simulink model "fft_inputs_equal_size_test"  (Simulink 7.2)
settings: Solver=VariableStepDiscrete  StartTime=0.0  StopTime=64  RelTol=1e-3
libraries: xbsIndex_r4 x249, casper_library_misc x24
(part 1 of 3)
settings Model: Creator=User  LastModifiedBy=root
settings OptimizationCC: InitFltsAndDblsToZero=on
settings DebuggingCC: SaveWithDisabledLinksMsg=none  SaveWithParameterizedLinksMsg=none

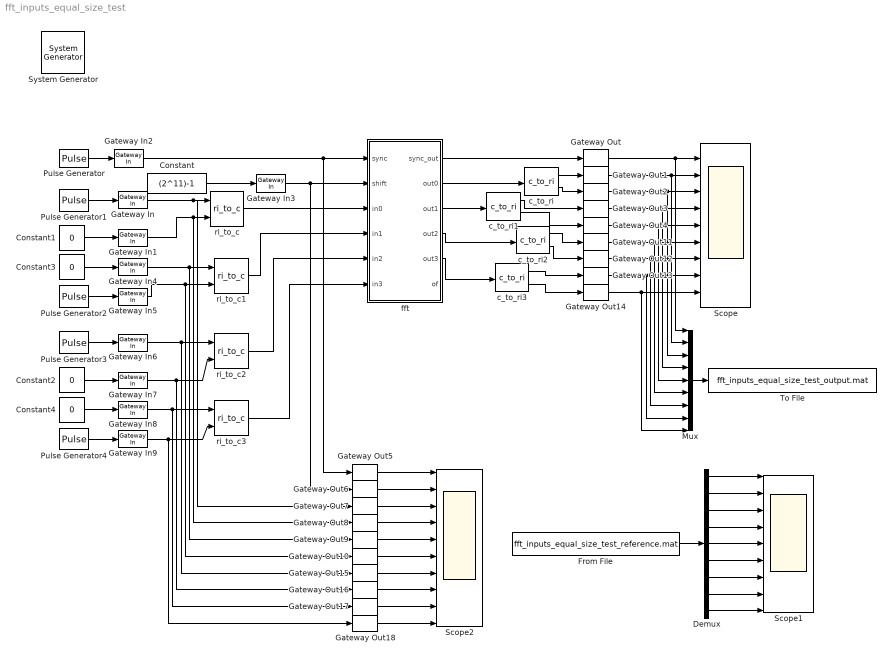
== system fft_inputs_equal_size_test ==
  " System Generator" : xbsIndex_r4/ System Generator  Tag=genX  SystemSampleTime=-1  xilinxfamily=Virtex4  part=xc4vsx35  speed=-10  package=ff668  synthesis_tool=XST  clock_wrapper=Clock Enables  directory=./netlist  testbench=off  simulink_period=1  sysclk_period=100  dcm_input_clock_period=100  incr_netlist=off  trim_vbits=Everywhere in SubSystem  dbl_ovrd=According to Block Masks  core_generation=According to Block Masks  run_coregen=off  deprecated_control=off  eval_field=0  block_type=sysgen
      settings: block_version=10.1.1
  Constant : Constant  Value=(2^11)-1  OutDataType=sfix(16)  OutScaling=2^0
  Constant{1..4} (4 alike) : Constant  Value=0  OutDataType=sfix(16)  OutScaling=2^0
  Demux : Demux  Outputs=9
  From File : FromFile  FileName=fft_inputs_equal_size_test_reference.mat  SampleTime=1
  Gateway In{,1,4..9} (8 alike) : xbsIndex_r4/Gateway In  arith_type="Signed  (2's comp)"  n_bits=8  bin_pt=7  quantization=Truncate  overflow=Wrap  period=1  dbl_ovrd=off  timing_constraint=None  locs_specified=off  LOCs={}  hdl_port=on  block_type=gatewayin
      settings: infoedit="Gateway in block.  Converts inputs of type Simulink integer, double and fixed point to  Xilinx fixed point type.<P><P>Hardware notes:  In hardware these blocks become top level input ports."  block_version=10.1.1
  Gateway In2 : xbsIndex_r4/Gateway In  arith_type=Boolean  n_bits=18  bin_pt=17  quantization=Truncate  overflow=Wrap  period=1  dbl_ovrd=off  timing_constraint=None  locs_specified=off  LOCs={}  hdl_port=on  block_type=gatewayin
      settings: infoedit="Gateway in block.  Converts inputs of type Simulink integer, double and fixed point to  Xilinx fixed point type.<P><P>Hardware notes:  In hardware these blocks become top level input ports."  block_version=10.1.1
  Gateway In3 : xbsIndex_r4/Gateway In  arith_type=Unsigned  n_bits=11  bin_pt=0  quantization=Truncate  overflow=Wrap  period=1  dbl_ovrd=off  timing_constraint=None  locs_specified=off  LOCs={}  hdl_port=on  block_type=gatewayin
      settings: infoedit="Gateway in block.  Converts inputs of type Simulink integer, double and fixed point to  Xilinx fixed point type.<P><P>Hardware notes:  In hardware these blocks become top level input ports."  block_version=10.1.1
  Gateway Out{,1..18} (19 alike) : xbsIndex_r4/Gateway Out  hdl_port=on  timing_constraint=None  locs_specified=off  LOCs={}  block_type=gatewayout
      settings: infoedit="Gateway out block.  Converts Xilinx fixed point inputs into ouputs of type Simulink integer, double, or fixed point.<P><P>Hardware notes:  In hardware these blocks become top level output ports or are discarded, depending on how they are configured."  block_version=10.1.1
  Mux : Mux  Inputs=9
  Pulse Generator : DiscretePulseGenerator  Period=2^4  PhaseDelay=11
  Pulse Generator1 : DiscretePulseGenerator  Period=2^2  PhaseDelay=13
  Pulse Generator2 : DiscretePulseGenerator  Period=2^3  PhaseDelay=13
  Pulse Generator3 : DiscretePulseGenerator  Period=2^2  PhaseDelay=13
  Pulse Generator4 : DiscretePulseGenerator  Period=2^3  PhaseDelay=13
  Scope : Scope  NumInputPorts=9
      settings: YMin=-1~0~0~-5~-5~-5~-5~-5~-5  YMax=2~1~1~5~5~5~5~5~5
  Scope1 : Scope  NumInputPorts=9
      settings: YMin=-1~0~0~-5~-5~-5~-5~-5~-5  YMax=2~1~1~5~5~5~5~5~5
  Scope2 : Scope  NumInputPorts=10
      settings: YMin=-1~0~0~-5~-5~-5~-5~-5~-5~-5  YMax=2~1~1~5~5~5~5~5~5~5  SaveName=ScopeData2
  To File : ToFile  Filename=fft_inputs_equal_size_test_output.mat  MatrixName=output
  c_to_ri{,1..3} (4 alike) : casper_library_misc/c_to_ri  SystemSampleTime=-1  n_bits=8  bin_pt=7
      settings: AttributesFormatString=8_7 r/i
  fft : Subsystem  AncestorBlock=casper_library_ffts/fft  mask(fft){FFTSize=2, input_bit_width=8, coeff_bit_width=8, n_inputs=2, quantization=Truncate, overflow=Wrap, add_latency=2, mult_latency=3, bram_latency=1, conv_latency=2, arch=Virtex2Pro, opt_target=multipliers, coeffs_bit_limit=8, delays_bit_limit=8, specify_mult=on, mult_spec=[1                                      2], dsp48_adders=off}
      mask prompts: FFTSize "Size of FFT: (2^?)"; input_bit_width "Input/Output Bit Width"; coeff_bit_width "Coefficient Bit Width"; n_inputs "Number of Simultaneous Inputs: (2^?)"; quantization "Quantization Behavior"; overflow "Overflow Behavior"; add_latency "Add Latency"; mult_latency "Mult Latency"; bram_latency "BRAM Latency"; conv_latency "Convert latency"; arch "Architecture"; opt_target "Use less"; coeffs_bit_limit "Number bits above which to store stage's coefficients in BRAM (2^? bits)"; delays_bit_limit "Number bits above which to store stage's delays in BRAM (2^? bits)"; specify_mult "Specify multiplier use (behavioral HDL if not specified)"; mult_spec "Multiplier specification (0=core, 1=embedded, 2=behavioural) (left=1st stage)"; dsp48_adders "DSP48 adders in butterfly"
      mask init:
      | fft_init(gcb,...
      |     'FFTSize', FFTSize, ...
      |     'input_bit_width', input_bit_width, ...
      |     'coeff_bit_width', coeff_bit_width, ...
      |     'n_inputs', n_inputs, ...
      |     'quantization', quantization, ...
      |     'overflow', overflow, ...
      |     'add_latency', add_latency, ...
      |     'mult_latency', mult_latency, ...
      |     'bram_latency', bram_latency, ...
      |     'conv_latency', conv_latency, ...
      |     'arch', arch, ...
      |     'opt_target', opt_target, ...
      |     'coeffs_bit_limit', coeffs_bit_limit, ...
      |     'delays_bit_limit', delays_bit_limit, ...
      |     'specify_mult', specify_mult, ...
      |     'mult_spec', mult_spec, ...
      |     'dsp48_adders', dsp48_adders);
      settings: AttributesFormatString=|
      | 2 stages
      | (8,8)
      | Truncate
      | Wrap
      mask Help: eval('xlWeb(''http://casper.berkeley.edu/wiki/Fft'')')
      mask StyleString: edit,edit,edit,edit,popup(Truncate|Round  (unbiased: +/- Inf)|Round  (unbiased: Even Values)),popup(Wrap|Saturate|Error),edit,edit,edit,edit,popup(Virtex2Pro|Virtex5),popup(logic|multipliers),edit,edit,checkbox,edit,checkbox
      mask CallbackString:
      | % fft_size = eval(get_param(gcb, 'FFTSize'));
      | % old_vec = eval(get_param(gcb, 'mult_spec'));
      | 
      | % vec = 2.*ones(1,fft_size);
      | % old_size = length(old_vec);
      | 
      | % if(old_size <= fft_size), size = old_size;
      | % else, size = fft_size;
      | % end
      | 
      | % for n = 1:size, vec(n) = old_vec(n); end
      | % set_param(gcb, 'mult_spec', mat2str(vec));||||||||||fft_callback_arch(gcb);||||specify_mult = get_param(gcb,'specify_mult');
      | visibs = get_param(gcb, 'MaskVisibilities');
      | if( strcmp(specify_mult,'off')), visibs{16} = 'off';
      | else visibs{16} = 'on';
      | end
      | set_param(gcb, 'MaskVisibilities', visibs);
      | 
      | |% vec = eval( get_param(gcb, 'mult_spec'));
      | % vec_size = length(vec);
      | % fft_size = eval( get_param(gcb, 'FFTSize'));
      | % new_vec = 2.*ones(1, fft_size);
      | 
      | % if(vec_size <= fft_size), size = vec_size;
      | % else size = fft_size;
      | % end
      | 
      | % for n=1:size,
      | %    new_vec(n) = vec(n);
      | % end
      | % set_param(gcb, 'mult_spec', mat2str(new_vec));|fft_callback_dsp48_adders(gcb);
  ri_to_c{,1..3} (4 alike) : casper_library_misc/ri_to_c  SystemSampleTime=-1
  wires:
  Pulse Generator/1 -> Gateway In2/1
  Gateway In2/1 -> Gateway Out5/1, fft/1(sync)
  Constant/1 -> Gateway In3/1
  Gateway In3/1 -> Gateway Out6/1, fft/2(shift)
  fft/1(sync_out) -> Gateway Out/1
  fft/2(out0) -> c_to_ri/1
  c_to_ri/1 -> Gateway Out1/1
  c_to_ri/2 -> Gateway Out2/1
  c_to_ri1/2 -> Gateway Out4/1
  fft/3(out1) -> c_to_ri1/1
  c_to_ri1/1 -> Gateway Out3/1
  Gateway Out/1 -> Scope/1, Mux/1
  Pulse Generator1/1 -> Gateway In/1
  Gateway In/1 -> ri_to_c/1, Gateway Out7/1
  Constant1/1 -> Gateway In1/1
  Gateway In1/1 -> ri_to_c/2, Gateway Out8/1
  Gateway In4/1 -> ri_to_c1/1, Gateway Out9/1
  Gateway In5/1 -> ri_to_c1/2, Gateway Out10/1
  Gateway Out1/1 -> Scope/2, Mux/2
  Gateway Out2/1 -> Scope/3, Mux/3
  Mux/1 -> To File/1
  Demux/1 -> Scope1/1
  Demux/2 -> Scope1/2
  Demux/3 -> Scope1/3
  Demux/4 -> Scope1/4
  Demux/5 -> Scope1/5
  Gateway Out5/1 -> Scope2/1
  Gateway Out6/1 -> Scope2/2
  Gateway Out7/1 -> Scope2/3
  Gateway Out8/1 -> Scope2/4
  Gateway Out9/1 -> Scope2/5
  Gateway Out10/1 -> Scope2/6
  Constant3/1 -> Gateway In4/1
  Pulse Generator2/1 -> Gateway In5/1
  Pulse Generator3/1 -> Gateway In6/1
  Constant2/1 -> Gateway In7/1
  Constant4/1 -> Gateway In8/1
  Pulse Generator4/1 -> Gateway In9/1
  Gateway In6/1 -> ri_to_c2/1, Gateway Out15/1
  Gateway In7/1 -> ri_to_c2/2, Gateway Out16/1
  Gateway In8/1 -> ri_to_c3/1, Gateway Out17/1
  Gateway In9/1 -> ri_to_c3/2, Gateway Out18/1
  ri_to_c/1 -> fft/3(in0)
  ri_to_c1/1 -> fft/4(in1)
  ri_to_c2/1 -> fft/5(in2)
  ri_to_c3/1 -> fft/6(in3)
  fft/4(out2) -> c_to_ri2/1
  fft/5(out3) -> c_to_ri3/1
  c_to_ri2/1 -> Gateway Out11/1
  c_to_ri2/2 -> Gateway Out12/1
  c_to_ri3/1 -> Gateway Out13/1
  c_to_ri3/2 -> Gateway Out14/1
  Gateway Out3/1 -> Scope/4, Mux/4
  Gateway Out4/1 -> Scope/5, Mux/5
  Gateway Out11/1 -> Scope/6, Mux/6
  Gateway Out12/1 -> Scope/7, Mux/7
  Gateway Out13/1 -> Scope/8, Mux/8
  Gateway Out14/1 -> Scope/9, Mux/9
  Gateway Out15/1 -> Scope2/7
  Gateway Out16/1 -> Scope2/8
  Gateway Out17/1 -> Scope2/9
  Gateway Out18/1 -> Scope2/10
  From File/1 -> Demux/1
  Demux/6 -> Scope1/6
  Demux/7 -> Scope1/7
  Demux/8 -> Scope1/8
  Demux/9 -> Scope1/9

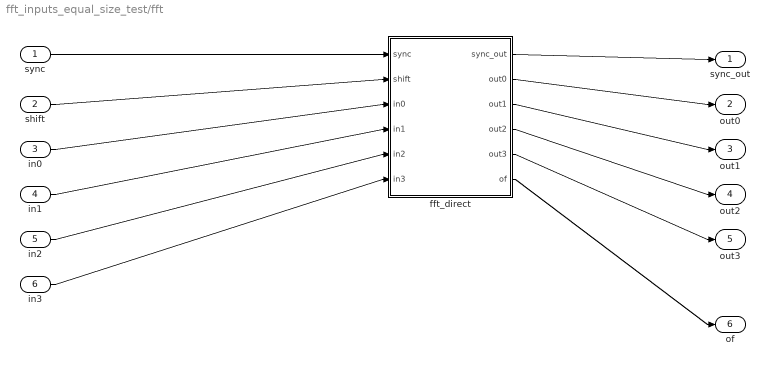
== system fft_inputs_equal_size_test/fft ==
  sync : Inport
  shift : Inport  Port=2
  in0 : Inport  Port=3
  in1 : Inport  Port=4
  in2 : Inport  Port=5
  in3 : Inport  Port=6
  fft_direct : Subsystem  AncestorBlock=casper_library_ffts/fft_direct  mask(fft_direct){FFTSize=2, input_bit_width=8, coeff_bit_width=8, add_latency=2, mult_latency=3, bram_latency=1, conv_latency=2, quantization=Truncate, overflow=Wrap, map_tail=off, LargerFFTSize=4, StartStage=4, arch=Virtex2Pro, opt_target=multipliers, coeffs_bit_limit=8, specify_mult=on, mult_spec=[1                                      2], dsp48_adders=off}
      mask prompts: FFTSize "Size of FFT: (2^?)"; input_bit_width "Input/Output Bit Width"; coeff_bit_width "Coefficient Bit Width"; add_latency "Add Latency"; mult_latency "Mult Latency"; bram_latency "BRAM Latency"; conv_latency "Convert latency"; quantization "Quantization Behavior"; overflow "Overflow Behavior"; map_tail "Map Tail of Larger FFT"; LargerFFTSize "Size of Larger FFT (2^?):"; StartStage "Start Stage of Map Tail:"; arch "Architecture"; opt_target "Use less"; coeffs_bit_limit "Number bits above which to store stage's coefficients in BRAM (2^? bits)"; specify_mult "Specify multiplier use (behavioural HDL if not specified)"; mult_spec "Multiplier specification (0=core, 1=behavioural HDL, 2=embedded) (left=1st stage)"; dsp48_adders "DSP48 adders in butterfly"
      mask help:
      | Implements an N-point FFT with the classic
      | butterfly structure with N inputs and N outputs
      mask init:
      | fft_direct_init(gcb,...
      |     'FFTSize', FFTSize, ...
      |     'input_bit_width', input_bit_width, ...
      |     'coeff_bit_width', coeff_bit_width, ...
      |     'add_latency', add_latency, ...
      |     'mult_latency', mult_latency, ...
      |     'bram_latency', bram_latency, ...
      |     'conv_latency', conv_latency, ...
      |     'quantization', quantization, ...
      |     'overflow', overflow, ...
      |     'map_tail', map_tail, ...
      |     'LargerFFTSize', LargerFFTSize, ...
      |     'StartStage', StartStage, ...
      |     'arch', arch, ...
      |     'opt_target', opt_target, ...
      |     'coeffs_bit_limit', coeffs_bit_limit, ...
      |     'specify_mult', specify_mult, ...
      |     'mult_spec', mult_spec, ...
      |     'dsp48_adders', dsp48_adders);
      settings: AttributesFormatString=|
      | Virtex2Pro
      | stages [4  5] of 2
      | [8,8]
      | Truncate
      | Wrap
      mask StyleString: edit,edit,edit,edit,edit,edit,edit,popup(Truncate|Round  (unbiased: +/- Inf)|Round  (unbiased: Even Values)),popup(Wrap|Saturate|Error),checkbox,edit,edit,popup(Virtex2Pro|Virtex5),popup(logic|multipliers),edit,checkbox,edit,checkbox
      mask CallbackString:
      | % fft_size = eval(get_param(gcb, 'FFTSize'));
      | % old_vec = eval(get_param(gcb, 'mult_spec'));
      | 
      | % vec = 2.*ones(1,fft_size);
      | % old_size = length(old_vec);
      | 
      | % if(old_size <= fft_size),
      | %     size = old_size;
      | % else,
      | %     size = fft_size;
      | % end
      | 
      | % for n = 1:size, vec(n) = old_vec(n); end
      | % set_param(gcb, 'mult_spec', mat2str(vec));|||||||||map_tail = get_param(gcb,'map_tail');
      | visibs = get_param(gcb, 'MaskVisibilities');
      | if( strcmp(map_tail,'off')),
      |     visibs{11} = 'off';
      |     visibs{12} = 'off';
      | else,
      |     visibs{11} = 'on';
      |     visibs{12} = 'on';
      | end
      | set_param(gcb, 'MaskVisibilities', visibs);
      | |||fft_callback_arch(gcb);|||specify_mult = get_param(gcb,'specify_mult');
      | visibs = get_param(gcb, 'MaskVisibilities');
      | if( strcmp(specify_mult,'off')), visibs{17} = 'off';
      | else, visibs{17} = 'on';
      | end
      | set_param(gcb, 'MaskVisibilities', visibs);
      | |% vec = eval( get_param(gcb, 'mult_spec'));
      | % vec_size = length(vec);
      | % fft_size = eval( get_param(gcb, 'FFTSize'));
      | % new_vec = 2.*ones(1, fft_size);
      | 
      | % if(vec_size <= fft_size), size = vec_size;
      | % else size = fft_size;
      | % end
      | 
      | % for n=1:size
      | %     new_vec(n) = vec(n);
      | % end
      | % set_param(gcb, 'mult_spec', mat2str(new_vec));|fft_callback_dsp48_adders(gcb);
  sync_out : Outport
  out0 : Outport  Port=2
  out1 : Outport  Port=3
  out2 : Outport  Port=4
  out3 : Outport  Port=5
  of : Outport  Port=6
  wires:
  sync/1 -> fft_direct/1(sync)
  shift/1 -> fft_direct/2(shift)
  fft_direct/1(sync_out) -> sync_out/1
  in0/1 -> fft_direct/3(in0)
  fft_direct/2(out0) -> out0/1
  in1/1 -> fft_direct/4(in1)
  fft_direct/3(out1) -> out1/1
  in2/1 -> fft_direct/5(in2)
  fft_direct/4(out2) -> out2/1
  in3/1 -> fft_direct/6(in3)
  fft_direct/5(out3) -> out3/1
  fft_direct/6(of) -> of/1

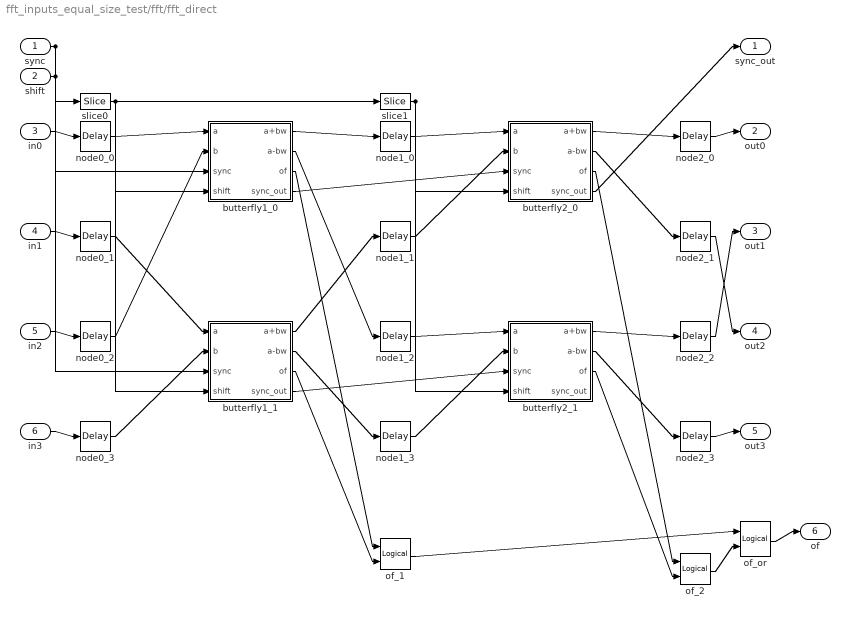
== system fft_inputs_equal_size_test/fft/fft_direct ==
  sync : Inport
  shift : Inport  Port=2
  in0 : Inport  Port=3
  in1 : Inport  Port=4
  in2 : Inport  Port=5
  in3 : Inport  Port=6
  butterfly1_0 : Subsystem  AncestorBlock=casper_library_ffts/butterfly_direct  mask(butterfly_direct){biplex=off, FFTSize=2, Coeffs=0, StepPeriod=0, coeffs_bram=off, coeff_bit_width=8, input_bit_width=8, bram_latency=1, add_latency=2, mult_latency=3, conv_latency=2, quantization=Truncate, overflow=Wrap, arch=Virtex2Pro, opt_target=multipliers, use_hdl=off, use_embedded=on, dsp48_adders=off}
      mask prompts: biplex "Used in biplex FFT"; FFTSize "Size of FFT: (2^?)"; Coeffs "Coefficients: (0 to 2^(FFTSize-1)-1)"; StepPeriod "Coefficient Step Period: (2^?)"; coeffs_bram "Implement coefficients in BRAM"; coeff_bit_width "Coefficient Bit Width"; input_bit_width "Input/Output Bit Width:"; bram_latency "BRAM Latency"; add_latency "Add Latency"; mult_latency "Mult Latency"; conv_latency "Convert latency"; quantization "Quantization Behavior"; overflow "Overflow Behavior"; arch "Architecture"; opt_target "Use less"; use_hdl "Use behavioural HDL for multipliers"; use_embedded "Use embedded multipliers"; dsp48_adders "Use DSP48s for adders"
      mask init:
      | butterfly_direct_init(gcb,...
      |     'biplex', biplex,...
      |     'FFTSize', FFTSize,...
      |     'Coeffs', Coeffs,...
      |     'coeff_bit_width', coeff_bit_width,...
      |     'StepPeriod', StepPeriod,...
      |     'input_bit_width', input_bit_width,...
      |     'add_latency', add_latency,...
      |     'mult_latency', mult_latency,...
      |     'bram_latency', bram_latency,...
      |     'conv_latency', conv_latency, ...
      |     'coeffs_bram', coeffs_bram,...    
      |     'quantization', quantization,...
      |     'overflow', overflow,...
      |     'arch', arch,...
      |     'opt_target', opt_target,...
      |     'use_hdl', use_hdl,...
      |     'use_embedded', use_embedded,...
      |     'dsp48_adders', dsp48_adders);
      settings: AttributesFormatString=|
      | twiddle_coeff_0
      | coeffs in slices
      mask StyleString: checkbox,edit,edit,edit,checkbox,edit,edit,edit,edit,edit,edit,popup(Truncate|Round  (unbiased: +/- Inf)|Round  (unbiased: Even Values)),popup(Wrap|Saturate|Error),popup(Virtex2Pro|Virtex5),popup(logic|multipliers),checkbox,checkbox,checkbox
      mask CallbackString:
      | ||%coeffs = eval(get_param(gcb,'Coeffs'));
      | %visibs = get_param(gcb,'MaskVisibilities');
      | %if length(coeffs) == 1,
      | %    visibs{4} = 'off'; visibs{5} = 'off';
      | %    visibs{6} = 'off';
      | %else
      | %    visibs{4} = 'on';
      | %    visibs{5} = 'on'; visibs{6} = 'on';
      | %end
      | %set_param(gcb, 'MaskVisibilities', visibs);|%coeffs = eval(get_param(gcb,'Coeffs'));
      | %visibs = get_param(gcb,'MaskVisibilities');
      | %if length(coeffs) == 1,
      | %    visibs{4} = 'off'; visibs{5} = 'off';
      | %    visibs{6} = 'off';
      | %else
      | %%    visibs{4} = 'on';
      | %    visibs{5} = 'on'; visibs{6} = 'on';
      | %end
      | %set_param(gcb, 'MaskVisibilities', visibs);|%coeffs = eval(get_param(gcb,'Coeffs'));
      | %visibs = get_param(gcb,'MaskVisibilities');
      | %if length(coeffs) == 1,
      | %    visibs{5} = 'off'; visibs{6} = 'off';
      | %    visibs{7} = 'off';
      | %else
      | %    visibs{5} = 'on';
      | %    visibs{6} = 'on'; visibs{7} = 'on';
      | %end
      | %set_param(gcb, 'MaskVisibilities', visibs);|||||||||fft_callback_arch(gcb);||use_hdl = get_param(gcb,'use_hdl');
      | visibs = get_param(gcb, 'MaskVisibilities');
      | if( strcmp(use_hdl,'on')),
      |     set_param(gcb, 'use_embedded','off');
      |     visibs{17} = 'off';
      | else,
      |     visibs{17} = 'on';
      | end
      |     set_param(gcb, 'MaskVisibilities',visibs);||fft_callback_dsp48_adders(gcb);
  butterfly1_1 : Subsystem  AncestorBlock=casper_library_ffts/butterfly_direct  mask(butterfly_direct){biplex=off, FFTSize=2, Coeffs=0, StepPeriod=0, coeffs_bram=off, coeff_bit_width=8, input_bit_width=8, bram_latency=1, add_latency=2, mult_latency=3, conv_latency=2, quantization=Truncate, overflow=Wrap, arch=Virtex2Pro, opt_target=multipliers, use_hdl=off, use_embedded=on, dsp48_adders=off}
      mask prompts: biplex "Used in biplex FFT"; FFTSize "Size of FFT: (2^?)"; Coeffs "Coefficients: (0 to 2^(FFTSize-1)-1)"; StepPeriod "Coefficient Step Period: (2^?)"; coeffs_bram "Implement coefficients in BRAM"; coeff_bit_width "Coefficient Bit Width"; input_bit_width "Input/Output Bit Width:"; bram_latency "BRAM Latency"; add_latency "Add Latency"; mult_latency "Mult Latency"; conv_latency "Convert latency"; quantization "Quantization Behavior"; overflow "Overflow Behavior"; arch "Architecture"; opt_target "Use less"; use_hdl "Use behavioural HDL for multipliers"; use_embedded "Use embedded multipliers"; dsp48_adders "Use DSP48s for adders"
      mask init: same as fft_inputs_equal_size_test/fft/fft_direct/butterfly1_0
      settings: AttributesFormatString=|
      | twiddle_coeff_0
      | coeffs in slices
      mask StyleString: checkbox,edit,edit,edit,checkbox,edit,edit,edit,edit,edit,edit,popup(Truncate|Round  (unbiased: +/- Inf)|Round  (unbiased: Even Values)),popup(Wrap|Saturate|Error),popup(Virtex2Pro|Virtex5),popup(logic|multipliers),checkbox,checkbox,checkbox
      mask CallbackString:
      | ||%coeffs = eval(get_param(gcb,'Coeffs'));
      | %visibs = get_param(gcb,'MaskVisibilities');
      | %if length(coeffs) == 1,
      | %    visibs{4} = 'off'; visibs{5} = 'off';
      | %    visibs{6} = 'off';
      | %else
      | %    visibs{4} = 'on';
      | %    visibs{5} = 'on'; visibs{6} = 'on';
      | %end
      | %set_param(gcb, 'MaskVisibilities', visibs);|%coeffs = eval(get_param(gcb,'Coeffs'));
      | %visibs = get_param(gcb,'MaskVisibilities');
      | %if length(coeffs) == 1,
      | %    visibs{4} = 'off'; visibs{5} = 'off';
      | %    visibs{6} = 'off';
      | %else
      | %%    visibs{4} = 'on';
      | %    visibs{5} = 'on'; visibs{6} = 'on';
      | %end
      | %set_param(gcb, 'MaskVisibilities', visibs);|%coeffs = eval(get_param(gcb,'Coeffs'));
      | %visibs = get_param(gcb,'MaskVisibilities');
      | %if length(coeffs) == 1,
      | %    visibs{5} = 'off'; visibs{6} = 'off';
      | %    visibs{7} = 'off';
      | %else
      | %    visibs{5} = 'on';
      | %    visibs{6} = 'on'; visibs{7} = 'on';
      | %end
      | %set_param(gcb, 'MaskVisibilities', visibs);|||||||||fft_callback_arch(gcb);||use_hdl = get_param(gcb,'use_hdl');
      | visibs = get_param(gcb, 'MaskVisibilities');
      | if( strcmp(use_hdl,'on')),
      |     set_param(gcb, 'use_embedded','off');
      |     visibs{17} = 'off';
      | else,
      |     visibs{17} = 'on';
      | end
      |     set_param(gcb, 'MaskVisibilities',visibs);||fft_callback_dsp48_adders(gcb);
  butterfly2_0 : Subsystem  AncestorBlock=casper_library_ffts/butterfly_direct  mask(butterfly_direct){biplex=off, FFTSize=2, Coeffs=0, StepPeriod=0, coeffs_bram=off, coeff_bit_width=8, input_bit_width=8, bram_latency=1, add_latency=2, mult_latency=3, conv_latency=2, quantization=Truncate, overflow=Wrap, arch=Virtex2Pro, opt_target=multipliers, use_hdl=on, use_embedded=off, dsp48_adders=off}
      mask prompts: biplex "Used in biplex FFT"; FFTSize "Size of FFT: (2^?)"; Coeffs "Coefficients: (0 to 2^(FFTSize-1)-1)"; StepPeriod "Coefficient Step Period: (2^?)"; coeffs_bram "Implement coefficients in BRAM"; coeff_bit_width "Coefficient Bit Width"; input_bit_width "Input/Output Bit Width:"; bram_latency "BRAM Latency"; add_latency "Add Latency"; mult_latency "Mult Latency"; conv_latency "Convert latency"; quantization "Quantization Behavior"; overflow "Overflow Behavior"; arch "Architecture"; opt_target "Use less"; use_hdl "Use behavioural HDL for multipliers"; use_embedded "Use embedded multipliers"; dsp48_adders "Use DSP48s for adders"
      mask init: same as fft_inputs_equal_size_test/fft/fft_direct/butterfly1_0
      settings: AttributesFormatString=|
      | twiddle_coeff_0
      | coeffs in slices
      mask StyleString: checkbox,edit,edit,edit,checkbox,edit,edit,edit,edit,edit,edit,popup(Truncate|Round  (unbiased: +/- Inf)|Round  (unbiased: Even Values)),popup(Wrap|Saturate|Error),popup(Virtex2Pro|Virtex5),popup(logic|multipliers),checkbox,checkbox,checkbox
      mask CallbackString:
      | ||%coeffs = eval(get_param(gcb,'Coeffs'));
      | %visibs = get_param(gcb,'MaskVisibilities');
      | %if length(coeffs) == 1,
      | %    visibs{4} = 'off'; visibs{5} = 'off';
      | %    visibs{6} = 'off';
      | %else
      | %    visibs{4} = 'on';
      | %    visibs{5} = 'on'; visibs{6} = 'on';
      | %end
      | %set_param(gcb, 'MaskVisibilities', visibs);|%coeffs = eval(get_param(gcb,'Coeffs'));
      | %visibs = get_param(gcb,'MaskVisibilities');
      | %if length(coeffs) == 1,
      | %    visibs{4} = 'off'; visibs{5} = 'off';
      | %    visibs{6} = 'off';
      | %else
      | %%    visibs{4} = 'on';
      | %    visibs{5} = 'on'; visibs{6} = 'on';
      | %end
      | %set_param(gcb, 'MaskVisibilities', visibs);|%coeffs = eval(get_param(gcb,'Coeffs'));
      | %visibs = get_param(gcb,'MaskVisibilities');
      | %if length(coeffs) == 1,
      | %    visibs{5} = 'off'; visibs{6} = 'off';
      | %    visibs{7} = 'off';
      | %else
      | %    visibs{5} = 'on';
      | %    visibs{6} = 'on'; visibs{7} = 'on';
      | %end
      | %set_param(gcb, 'MaskVisibilities', visibs);|||||||||fft_callback_arch(gcb);||use_hdl = get_param(gcb,'use_hdl');
      | visibs = get_param(gcb, 'MaskVisibilities');
      | if( strcmp(use_hdl,'on')),
      |     set_param(gcb, 'use_embedded','off');
      |     visibs{17} = 'off';
      | else,
      |     visibs{17} = 'on';
      | end
      |     set_param(gcb, 'MaskVisibilities',visibs);||fft_callback_dsp48_adders(gcb);
  butterfly2_1 : Subsystem  AncestorBlock=casper_library_ffts/butterfly_direct  mask(butterfly_direct){biplex=off, FFTSize=2, Coeffs=1, StepPeriod=0, coeffs_bram=off, coeff_bit_width=8, input_bit_width=8, bram_latency=1, add_latency=2, mult_latency=3, conv_latency=2, quantization=Truncate, overflow=Wrap, arch=Virtex2Pro, opt_target=multipliers, use_hdl=on, use_embedded=off, dsp48_adders=off}
      mask prompts: biplex "Used in biplex FFT"; FFTSize "Size of FFT: (2^?)"; Coeffs "Coefficients: (0 to 2^(FFTSize-1)-1)"; StepPeriod "Coefficient Step Period: (2^?)"; coeffs_bram "Implement coefficients in BRAM"; coeff_bit_width "Coefficient Bit Width"; input_bit_width "Input/Output Bit Width:"; bram_latency "BRAM Latency"; add_latency "Add Latency"; mult_latency "Mult Latency"; conv_latency "Convert latency"; quantization "Quantization Behavior"; overflow "Overflow Behavior"; arch "Architecture"; opt_target "Use less"; use_hdl "Use behavioural HDL for multipliers"; use_embedded "Use embedded multipliers"; dsp48_adders "Use DSP48s for adders"
      mask init: same as fft_inputs_equal_size_test/fft/fft_direct/butterfly1_0
      settings: AttributesFormatString=|
      | twiddle_coeff_1
      | coeffs in slices
      mask StyleString: checkbox,edit,edit,edit,checkbox,edit,edit,edit,edit,edit,edit,popup(Truncate|Round  (unbiased: +/- Inf)|Round  (unbiased: Even Values)),popup(Wrap|Saturate|Error),popup(Virtex2Pro|Virtex5),popup(logic|multipliers),checkbox,checkbox,checkbox
      mask CallbackString:
      | ||%coeffs = eval(get_param(gcb,'Coeffs'));
      | %visibs = get_param(gcb,'MaskVisibilities');
      | %if length(coeffs) == 1,
      | %    visibs{4} = 'off'; visibs{5} = 'off';
      | %    visibs{6} = 'off';
      | %else
      | %    visibs{4} = 'on';
      | %    visibs{5} = 'on'; visibs{6} = 'on';
      | %end
      | %set_param(gcb, 'MaskVisibilities', visibs);|%coeffs = eval(get_param(gcb,'Coeffs'));
      | %visibs = get_param(gcb,'MaskVisibilities');
      | %if length(coeffs) == 1,
      | %    visibs{4} = 'off'; visibs{5} = 'off';
      | %    visibs{6} = 'off';
      | %else
      | %%    visibs{4} = 'on';
      | %    visibs{5} = 'on'; visibs{6} = 'on';
      | %end
      | %set_param(gcb, 'MaskVisibilities', visibs);|%coeffs = eval(get_param(gcb,'Coeffs'));
      | %visibs = get_param(gcb,'MaskVisibilities');
      | %if length(coeffs) == 1,
      | %    visibs{5} = 'off'; visibs{6} = 'off';
      | %    visibs{7} = 'off';
      | %else
      | %    visibs{5} = 'on';
      | %    visibs{6} = 'on'; visibs{7} = 'on';
      | %end
      | %set_param(gcb, 'MaskVisibilities', visibs);|||||||||fft_callback_arch(gcb);||use_hdl = get_param(gcb,'use_hdl');
      | visibs = get_param(gcb, 'MaskVisibilities');
      | if( strcmp(use_hdl,'on')),
      |     set_param(gcb, 'use_embedded','off');
      |     visibs{17} = 'off';
      | else,
      |     visibs{17} = 'on';
      | end
      |     set_param(gcb, 'MaskVisibilities',visibs);||fft_callback_dsp48_adders(gcb);
  node0_{0..3} (4 alike) : xbsIndex_r4/Delay  en=off  latency=0  dbl_ovrd=off  reg_retiming=off  block_type=delay
      settings: block_version=11.4
  node1_{0..3} (4 alike) : xbsIndex_r4/Delay  en=off  latency=0  dbl_ovrd=off  reg_retiming=off  block_type=delay
      settings: block_version=11.4
  node2_{0..3} (4 alike) : xbsIndex_r4/Delay  en=off  latency=0  dbl_ovrd=off  reg_retiming=off  block_type=delay
      settings: block_version=11.4
  of_1 : xbsIndex_r4/Logical  logical_function=OR  inputs=2  en=off  latency=1  precision=Full  arith_type=Unsigned  n_bits=16  bin_pt=0  align_bp=on  dbl_ovrd=off  block_type=logical
      settings: block_version=11.4
  of_2 : xbsIndex_r4/Logical  logical_function=OR  inputs=2  en=off  latency=1  precision=Full  arith_type=Unsigned  n_bits=16  bin_pt=0  align_bp=on  dbl_ovrd=off  block_type=logical
      settings: block_version=11.4
  of_or : xbsIndex_r4/Logical  logical_function=OR  inputs=2  en=off  latency=0  precision=Full  arith_type=Unsigned  n_bits=16  bin_pt=0  align_bp=on  dbl_ovrd=off  block_type=logical
      settings: block_version=11.4
  slice0 : xbsIndex_r4/Slice  nbits=1  boolean_output=on  mode=Lower Bit Location + Width  bit1=0  base1=MSB of Input  bit0=0  base0=LSB of Input  dbl_ovrd=off  block_type=slice
  slice1 : xbsIndex_r4/Slice  nbits=1  boolean_output=on  mode=Lower Bit Location + Width  bit1=0  base1=MSB of Input  bit0=1  base0=LSB of Input  dbl_ovrd=off  block_type=slice
  sync_out : Outport
  out0 : Outport  Port=2
  out1 : Outport  Port=3
  out2 : Outport  Port=4
  out3 : Outport  Port=5
  of : Outport  Port=6
  wires:
  of_or/1 -> of/1
  in0/1 -> node0_0/1
  in1/1 -> node0_1/1
  in2/1 -> node0_2/1
  in3/1 -> node0_3/1
  shift/1 -> slice0/1, slice1/1
  node2_0/1 -> out0/1
  node2_1/1 -> out2/1
  node2_2/1 -> out1/1
  node2_3/1 -> out3/1
  of_1/1 -> of_or/1
  node0_0/1 -> butterfly1_0/1(a)
  node0_2/1 -> butterfly1_0/2(b)
  butterfly1_0/1(a+bw) -> node1_0/1
  butterfly1_0/2(a-bw) -> node1_2/1
  sync/1 -> butterfly1_0/3(sync), butterfly1_1/3(sync)
  slice0/1 -> butterfly1_0/4(shift), butterfly1_1/4(shift)
  butterfly1_0/3(of) -> of_1/1
  node0_1/1 -> butterfly1_1/1(a)
  node0_3/1 -> butterfly1_1/2(b)
  butterfly1_1/1(a+bw) -> node1_1/1
  butterfly1_1/2(a-bw) -> node1_3/1
  butterfly1_1/3(of) -> of_1/2
  of_2/1 -> of_or/2
  node1_0/1 -> butterfly2_0/1(a)
  node1_1/1 -> butterfly2_0/2(b)
  butterfly2_0/1(a+bw) -> node2_0/1
  butterfly2_0/2(a-bw) -> node2_1/1
  butterfly1_0/4(sync_out) -> butterfly2_0/3(sync)
  butterfly2_0/4(sync_out) -> sync_out/1
  slice1/1 -> butterfly2_0/4(shift), butterfly2_1/4(shift)
  butterfly2_0/3(of) -> of_2/1
  node1_2/1 -> butterfly2_1/1(a)
  node1_3/1 -> butterfly2_1/2(b)
  butterfly2_1/1(a+bw) -> node2_2/1
  butterfly2_1/2(a-bw) -> node2_3/1
  butterfly1_1/4(sync_out) -> butterfly2_1/3(sync)
  butterfly2_1/3(of) -> of_2/2

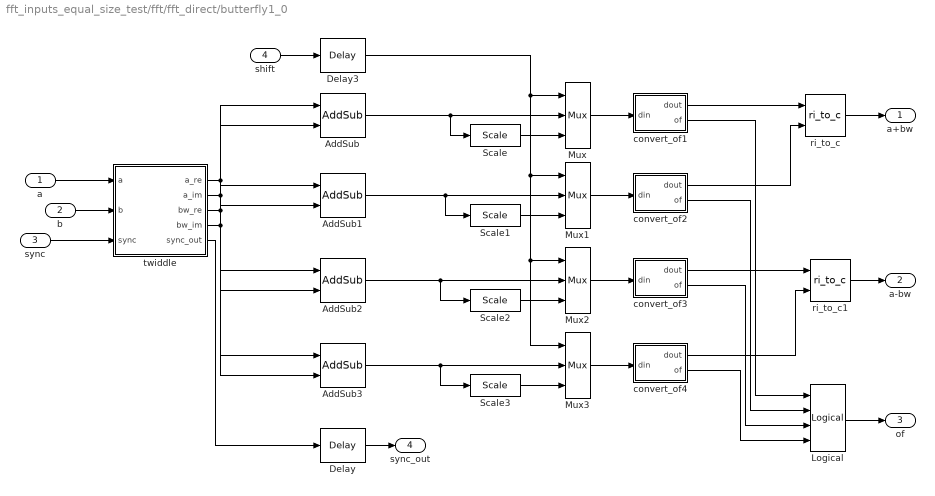
== system fft_inputs_equal_size_test/fft/fft_direct/butterfly1_0 ==
  a : Inport  OutDataType=sfix(16)  OutScaling=2^0
  b : Inport  Port=2  OutDataType=sfix(16)  OutScaling=2^0
  sync : Inport  Port=3  OutDataType=sfix(16)  OutScaling=2^0
  shift : Inport  Port=4  OutDataType=sfix(16)  OutScaling=2^0
  AddSub : xbsIndex_r4/AddSub  mode=Addition  use_carryin=off  use_carryout=off  en=off  latency=add_latency  precision=Full  arith_type=Unsigned  n_bits=8  bin_pt=2  quantization=Truncate  overflow=Wrap  dbl_ovrd=off  use_behavioral_HDL=on  hw_selection=DSP48  pipelined=on  use_rpm=on  block_type=addsub
      settings: xl_area=[0, 0, 0, 0, 0, 0, 0]  block_version=9.1.01
  AddSub1 : xbsIndex_r4/AddSub  mode=Addition  use_carryin=off  use_carryout=off  en=off  latency=add_latency  precision=Full  arith_type=Unsigned  n_bits=8  bin_pt=2  quantization=Truncate  overflow=Wrap  dbl_ovrd=off  use_behavioral_HDL=on  hw_selection=DSP48  pipelined=on  use_rpm=on  block_type=addsub
      settings: xl_area=[0, 0, 0, 0, 0, 0, 0]  block_version=9.1.01
  AddSub2 : xbsIndex_r4/AddSub  mode=Subtraction  use_carryin=off  use_carryout=off  en=off  latency=add_latency  precision=Full  arith_type=Unsigned  n_bits=8  bin_pt=2  quantization=Truncate  overflow=Wrap  dbl_ovrd=off  use_behavioral_HDL=on  hw_selection=DSP48  pipelined=on  use_rpm=on  block_type=addsub
      settings: xl_area=[0, 0, 0, 0, 0, 0, 0]  block_version=9.1.01
  AddSub3 : xbsIndex_r4/AddSub  mode=Subtraction  use_carryin=off  use_carryout=off  en=off  latency=add_latency  precision=Full  arith_type=Unsigned  n_bits=8  bin_pt=2  quantization=Truncate  overflow=Wrap  dbl_ovrd=off  use_behavioral_HDL=on  hw_selection=DSP48  pipelined=on  use_rpm=on  block_type=addsub
      settings: xl_area=[0, 0, 0, 0, 0, 0, 0]  block_version=9.1.01
  Delay : xbsIndex_r4/Delay  en=off  latency=add_latency + conv_latency + 1  dbl_ovrd=off  reg_retiming=on  block_type=delay
      settings: xl_area=[0, 0, 0, 0, 0, 0, 0]  block_version=9.1.01
  Delay3 : xbsIndex_r4/Delay  en=off  latency=add_latency  dbl_ovrd=off  reg_retiming=off  block_type=delay
      settings: xl_area=[0, 0, 0, 0, 0, 0, 0]  block_version=9.1.01
  Logical : xbsIndex_r4/Logical  logical_function=OR  inputs=4  en=off  latency=0  precision=Full  arith_type=Unsigned  n_bits=16  bin_pt=0  align_bp=on  dbl_ovrd=off  block_type=logical
      settings: block_version=10.1.1
  Mux{,1..3} (4 alike) : xbsIndex_r4/Mux  inputs=2  en=off  latency=1  precision=Full  arith_type="Signed  (2's comp)"  n_bits=8  bin_pt=2  quantization=Truncate  overflow=Wrap  dbl_ovrd=off  block_type=mux
      settings: xl_area=[0, 0, 0, 0, 0, 0, 0]  block_version=9.1.01
  Scale{,1..3} (4 alike) : xbsIndex_r4/Scale  scale_factor=-1  dbl_ovrd=off  block_type=scale
      settings: infoedit=Scales input by a power of two by adjusting the binary point position.<P><P>Hardware notes: In hardware this block costs nothing.  block_version=9.1.01
  convert_of1 : Subsystem  AncestorBlock=casper_library_misc/convert_of  mask(convert_of){bit_width_i=10, binary_point_i=8, bit_width_o=8, binary_point_o=7, latency=2, overflow=Wrap, quantization=Truncate}
      mask prompts: bit_width_i "Bit Width In"; binary_point_i "Binary Point In"; bit_width_o "Bit Width Out"; binary_point_o "Binary Point Out"; overflow "Overflow Behaviour"; quantization "Quantization Behaviour"
      mask help:
      | Converts from one 2's complement bit-width
      | and/or binary point position to another.
      | Includes underflow/overflow indicator.
      mask init:
      | convert_of_init(gcb, ...
      |     'bit_width_i', bit_width_i, ...
      |     'binary_point_i', binary_point_i, ...
      |     'bit_width_o', bit_width_o, ...
      |     'binary_point_o', binary_point_o, ...
      |     'latency', latency, ...
      |     'overflow', overflow, ...
      |     'quantization', quantization);
      settings: AttributesFormatString=[10,8]->[8,7]
      mask StyleString: edit,edit,edit,edit,edit,popup(Wrap|Saturate|Error),popup(Truncate|Round  (unbiased: +/- Inf)|Round  (unbiased: even values))
  convert_of2 : Subsystem  AncestorBlock=casper_library_misc/convert_of  mask(convert_of){bit_width_i=10, binary_point_i=8, bit_width_o=8, binary_point_o=7, latency=2, overflow=Wrap, quantization=Truncate}
      mask prompts: bit_width_i "Bit Width In"; binary_point_i "Binary Point In"; bit_width_o "Bit Width Out"; binary_point_o "Binary Point Out"; overflow "Overflow Behaviour"; quantization "Quantization Behaviour"
      mask help:
      | Converts from one 2's complement bit-width
      | and/or binary point position to another.
      | Includes underflow/overflow indicator.
      mask init: same as fft_inputs_equal_size_test/fft/fft_direct/butterfly1_0/convert_of1
      settings: AttributesFormatString=[10,8]->[8,7]
      mask StyleString: edit,edit,edit,edit,edit,popup(Wrap|Saturate|Error),popup(Truncate|Round  (unbiased: +/- Inf)|Round  (unbiased: even values))
  convert_of3 : Subsystem  AncestorBlock=casper_library_misc/convert_of  mask(convert_of){bit_width_i=10, binary_point_i=8, bit_width_o=8, binary_point_o=7, latency=2, overflow=Wrap, quantization=Truncate}
      mask prompts: bit_width_i "Bit Width In"; binary_point_i "Binary Point In"; bit_width_o "Bit Width Out"; binary_point_o "Binary Point Out"; overflow "Overflow Behaviour"; quantization "Quantization Behaviour"
      mask help:
      | Converts from one 2's complement bit-width
      | and/or binary point position to another.
      | Includes underflow/overflow indicator.
      mask init: same as fft_inputs_equal_size_test/fft/fft_direct/butterfly1_0/convert_of1
      settings: AttributesFormatString=[10,8]->[8,7]
      mask StyleString: edit,edit,edit,edit,edit,popup(Wrap|Saturate|Error),popup(Truncate|Round  (unbiased: +/- Inf)|Round  (unbiased: even values))
  convert_of4 : Subsystem  AncestorBlock=casper_library_misc/convert_of  mask(convert_of){bit_width_i=10, binary_point_i=8, bit_width_o=8, binary_point_o=7, latency=2, overflow=Wrap, quantization=Truncate}
      mask prompts: bit_width_i "Bit Width In"; binary_point_i "Binary Point In"; bit_width_o "Bit Width Out"; binary_point_o "Binary Point Out"; overflow "Overflow Behaviour"; quantization "Quantization Behaviour"
      mask help:
      | Converts from one 2's complement bit-width
      | and/or binary point position to another.
      | Includes underflow/overflow indicator.
      mask init: same as fft_inputs_equal_size_test/fft/fft_direct/butterfly1_0/convert_of1
      settings: AttributesFormatString=[10,8]->[8,7]
      mask StyleString: edit,edit,edit,edit,edit,popup(Wrap|Saturate|Error),popup(Truncate|Round  (unbiased: +/- Inf)|Round  (unbiased: even values))
  ri_to_c : casper_library_misc/ri_to_c  SystemSampleTime=-1
  ri_to_c1 : casper_library_misc/ri_to_c  SystemSampleTime=-1
  twiddle : Subsystem  AncestorBlock=casper_library_ffts_twiddle/twiddle_coeff_0  mask(twiddle_coeff_0){FFTSize=2, input_bit_width=8, add_latency=2, mult_latency=3, bram_latency=1, conv_latency=2, opt_target=multipliers}
      mask prompts: FFTSize "FFT Size (2^?)"; input_bit_width "Input Bit Width"; add_latency "Add Latency"; mult_latency "Mult Latency"; bram_latency "BRAM Latency"; conv_latency "Convert latency"; opt_target "Use less"
      mask help:
      | Used in FFT library. Used when coefficients
      | are 2^0 (just pass data through) but latency
      | must be the same as for a full twiddle.
      mask init:
      | set_param(gcb,'LinkStatus','inactive');
      | if(strcmp(opt_target, 'logic')), 
      |     latency = 'mult_latency+add_latency+bram_latency+conv_latency';
      | else,
      |     latency = 'mult_latency+add_latency*2+bram_latency+conv_latency';
      | end
      | set_param([gcb,'/delay0'], 'latency', latency);
      | set_param([gcb,'/delay1'], 'latency', latency);
      | set_param([gcb,'/delay2'], 'latency', latency);
      mask StyleString: edit,edit,edit,edit,edit,edit,popup(logic|multipliers)
  a+bw : Outport  OutDataType=sfix(16)  OutScaling=2^0
  a-bw : Outport  Port=2  OutDataType=sfix(16)  OutScaling=2^0
  of : Outport  Port=3  OutDataType=sfix(16)  OutScaling=2^0
  sync_out : Outport  Port=4  OutDataType=sfix(16)  OutScaling=2^0
  wires:
  convert_of4/2(of) -> Logical/4
  convert_of3/2(of) -> Logical/3
  convert_of2/2(of) -> Logical/2
  convert_of1/2(of) -> Logical/1
  convert_of4/1(dout) -> ri_to_c1/2
  Mux3/1 -> convert_of4/1(din)
  AddSub3/1 -> Scale3/1, Mux3/2
  Scale3/1 -> Mux3/3
  convert_of3/1(dout) -> ri_to_c1/1
  Mux2/1 -> convert_of3/1(din)
  AddSub2/1 -> Scale2/1, Mux2/2
  Scale2/1 -> Mux2/3
  convert_of2/1(dout) -> ri_to_c/2
  Mux1/1 -> convert_of2/1(din)
  AddSub1/1 -> Scale1/1, Mux1/2
  Scale1/1 -> Mux1/3
  convert_of1/1(dout) -> ri_to_c/1
  Mux/1 -> convert_of1/1(din)
  twiddle/4(bw_im) -> AddSub3/2, AddSub1/2
  twiddle/3(bw_re) -> AddSub2/2, AddSub/2
  twiddle/2(a_im) -> AddSub3/1, AddSub1/1
  twiddle/1(a_re) -> AddSub2/1, AddSub/1
  sync/1 -> twiddle/3(sync)
  b/1 -> twiddle/2(b)
  a/1 -> twiddle/1(a)
  ri_to_c/1 -> a+bw/1
  ri_to_c1/1 -> a-bw/1
  Delay/1 -> sync_out/1
  AddSub/1 -> Mux/2, Scale/1
  shift/1 -> Delay3/1
  Scale/1 -> Mux/3
  Delay3/1 -> Mux3/1, Mux2/1, Mux1/1, Mux/1
  Logical/1 -> of/1
  twiddle/5(sync_out) -> Delay/1

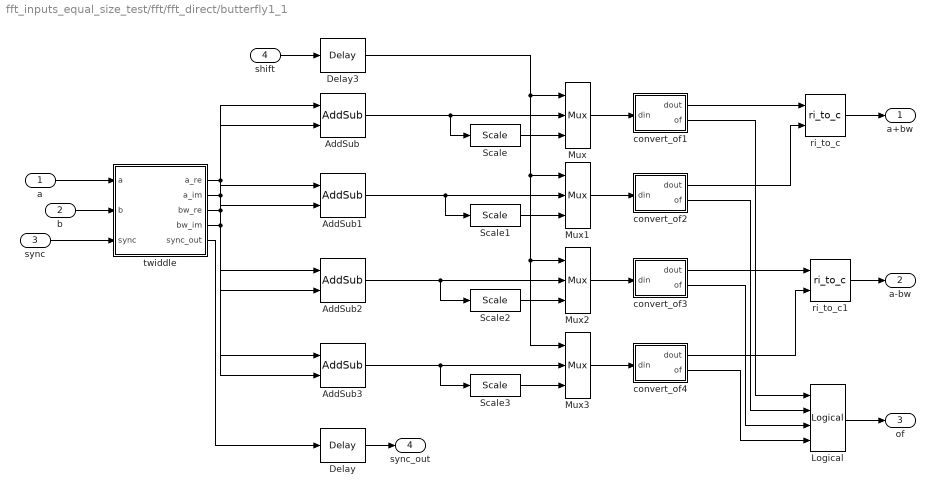
== system fft_inputs_equal_size_test/fft/fft_direct/butterfly1_1 ==
  a : Inport  OutDataType=sfix(16)  OutScaling=2^0
  b : Inport  Port=2  OutDataType=sfix(16)  OutScaling=2^0
  sync : Inport  Port=3  OutDataType=sfix(16)  OutScaling=2^0
  shift : Inport  Port=4  OutDataType=sfix(16)  OutScaling=2^0
  AddSub : xbsIndex_r4/AddSub  mode=Addition  use_carryin=off  use_carryout=off  en=off  latency=add_latency  precision=Full  arith_type=Unsigned  n_bits=8  bin_pt=2  quantization=Truncate  overflow=Wrap  dbl_ovrd=off  use_behavioral_HDL=on  hw_selection=DSP48  pipelined=on  use_rpm=on  block_type=addsub
      settings: xl_area=[0, 0, 0, 0, 0, 0, 0]  block_version=9.1.01
  AddSub1 : xbsIndex_r4/AddSub  mode=Addition  use_carryin=off  use_carryout=off  en=off  latency=add_latency  precision=Full  arith_type=Unsigned  n_bits=8  bin_pt=2  quantization=Truncate  overflow=Wrap  dbl_ovrd=off  use_behavioral_HDL=on  hw_selection=DSP48  pipelined=on  use_rpm=on  block_type=addsub
      settings: xl_area=[0, 0, 0, 0, 0, 0, 0]  block_version=9.1.01
  AddSub2 : xbsIndex_r4/AddSub  mode=Subtraction  use_carryin=off  use_carryout=off  en=off  latency=add_latency  precision=Full  arith_type=Unsigned  n_bits=8  bin_pt=2  quantization=Truncate  overflow=Wrap  dbl_ovrd=off  use_behavioral_HDL=on  hw_selection=DSP48  pipelined=on  use_rpm=on  block_type=addsub
      settings: xl_area=[0, 0, 0, 0, 0, 0, 0]  block_version=9.1.01
  AddSub3 : xbsIndex_r4/AddSub  mode=Subtraction  use_carryin=off  use_carryout=off  en=off  latency=add_latency  precision=Full  arith_type=Unsigned  n_bits=8  bin_pt=2  quantization=Truncate  overflow=Wrap  dbl_ovrd=off  use_behavioral_HDL=on  hw_selection=DSP48  pipelined=on  use_rpm=on  block_type=addsub
      settings: xl_area=[0, 0, 0, 0, 0, 0, 0]  block_version=9.1.01
  Delay : xbsIndex_r4/Delay  en=off  latency=add_latency + conv_latency + 1  dbl_ovrd=off  reg_retiming=on  block_type=delay
      settings: xl_area=[0, 0, 0, 0, 0, 0, 0]  block_version=9.1.01
  Delay3 : xbsIndex_r4/Delay  en=off  latency=add_latency  dbl_ovrd=off  reg_retiming=off  block_type=delay
      settings: xl_area=[0, 0, 0, 0, 0, 0, 0]  block_version=9.1.01
  Logical : xbsIndex_r4/Logical  logical_function=OR  inputs=4  en=off  latency=0  precision=Full  arith_type=Unsigned  n_bits=16  bin_pt=0  align_bp=on  dbl_ovrd=off  block_type=logical
      settings: block_version=10.1.1
  Mux{,1..3} (4 alike) : xbsIndex_r4/Mux  inputs=2  en=off  latency=1  precision=Full  arith_type="Signed  (2's comp)"  n_bits=8  bin_pt=2  quantization=Truncate  overflow=Wrap  dbl_ovrd=off  block_type=mux
      settings: xl_area=[0, 0, 0, 0, 0, 0, 0]  block_version=9.1.01
  Scale{,1..3} (4 alike) : xbsIndex_r4/Scale  scale_factor=-1  dbl_ovrd=off  block_type=scale
      settings: infoedit=Scales input by a power of two by adjusting the binary point position.<P><P>Hardware notes: In hardware this block costs nothing.  block_version=9.1.01
  convert_of1 : Subsystem  AncestorBlock=casper_library_misc/convert_of  mask(convert_of){bit_width_i=10, binary_point_i=8, bit_width_o=8, binary_point_o=7, latency=2, overflow=Wrap, quantization=Truncate}
      mask prompts: bit_width_i "Bit Width In"; binary_point_i "Binary Point In"; bit_width_o "Bit Width Out"; binary_point_o "Binary Point Out"; overflow "Overflow Behaviour"; quantization "Quantization Behaviour"
      mask help:
      | Converts from one 2's complement bit-width
      | and/or binary point position to another.
      | Includes underflow/overflow indicator.
      mask init: same as fft_inputs_equal_size_test/fft/fft_direct/butterfly1_0/convert_of1
      settings: AttributesFormatString=[10,8]->[8,7]
      mask StyleString: edit,edit,edit,edit,edit,popup(Wrap|Saturate|Error),popup(Truncate|Round  (unbiased: +/- Inf)|Round  (unbiased: even values))
  convert_of2 : Subsystem  AncestorBlock=casper_library_misc/convert_of  mask(convert_of){bit_width_i=10, binary_point_i=8, bit_width_o=8, binary_point_o=7, latency=2, overflow=Wrap, quantization=Truncate}
      mask prompts: bit_width_i "Bit Width In"; binary_point_i "Binary Point In"; bit_width_o "Bit Width Out"; binary_point_o "Binary Point Out"; overflow "Overflow Behaviour"; quantization "Quantization Behaviour"
      mask help:
      | Converts from one 2's complement bit-width
      | and/or binary point position to another.
      | Includes underflow/overflow indicator.
      mask init: same as fft_inputs_equal_size_test/fft/fft_direct/butterfly1_0/convert_of1
      settings: AttributesFormatString=[10,8]->[8,7]
      mask StyleString: edit,edit,edit,edit,edit,popup(Wrap|Saturate|Error),popup(Truncate|Round  (unbiased: +/- Inf)|Round  (unbiased: even values))
  convert_of3 : Subsystem  AncestorBlock=casper_library_misc/convert_of  mask(convert_of){bit_width_i=10, binary_point_i=8, bit_width_o=8, binary_point_o=7, latency=2, overflow=Wrap, quantization=Truncate}
      mask prompts: bit_width_i "Bit Width In"; binary_point_i "Binary Point In"; bit_width_o "Bit Width Out"; binary_point_o "Binary Point Out"; overflow "Overflow Behaviour"; quantization "Quantization Behaviour"
      mask help:
      | Converts from one 2's complement bit-width
      | and/or binary point position to another.
      | Includes underflow/overflow indicator.
      mask init: same as fft_inputs_equal_size_test/fft/fft_direct/butterfly1_0/convert_of1
      settings: AttributesFormatString=[10,8]->[8,7]
      mask StyleString: edit,edit,edit,edit,edit,popup(Wrap|Saturate|Error),popup(Truncate|Round  (unbiased: +/- Inf)|Round  (unbiased: even values))
  convert_of4 : Subsystem  AncestorBlock=casper_library_misc/convert_of  mask(convert_of){bit_width_i=10, binary_point_i=8, bit_width_o=8, binary_point_o=7, latency=2, overflow=Wrap, quantization=Truncate}
      mask prompts: bit_width_i "Bit Width In"; binary_point_i "Binary Point In"; bit_width_o "Bit Width Out"; binary_point_o "Binary Point Out"; overflow "Overflow Behaviour"; quantization "Quantization Behaviour"
      mask help:
      | Converts from one 2's complement bit-width
      | and/or binary point position to another.
      | Includes underflow/overflow indicator.
      mask init: same as fft_inputs_equal_size_test/fft/fft_direct/butterfly1_0/convert_of1
      settings: AttributesFormatString=[10,8]->[8,7]
      mask StyleString: edit,edit,edit,edit,edit,popup(Wrap|Saturate|Error),popup(Truncate|Round  (unbiased: +/- Inf)|Round  (unbiased: even values))
  ri_to_c : casper_library_misc/ri_to_c  SystemSampleTime=-1
  ri_to_c1 : casper_library_misc/ri_to_c  SystemSampleTime=-1
  twiddle : Subsystem  AncestorBlock=casper_library_ffts_twiddle/twiddle_coeff_0  mask(twiddle_coeff_0){FFTSize=2, input_bit_width=8, add_latency=2, mult_latency=3, bram_latency=1, conv_latency=2, opt_target=multipliers}
      mask prompts: FFTSize "FFT Size (2^?)"; input_bit_width "Input Bit Width"; add_latency "Add Latency"; mult_latency "Mult Latency"; bram_latency "BRAM Latency"; conv_latency "Convert latency"; opt_target "Use less"
      mask help:
      | Used in FFT library. Used when coefficients
      | are 2^0 (just pass data through) but latency
      | must be the same as for a full twiddle.
      mask init: same as fft_inputs_equal_size_test/fft/fft_direct/butterfly1_0/twiddle
      mask StyleString: edit,edit,edit,edit,edit,edit,popup(logic|multipliers)
  a+bw : Outport  OutDataType=sfix(16)  OutScaling=2^0
  a-bw : Outport  Port=2  OutDataType=sfix(16)  OutScaling=2^0
  of : Outport  Port=3  OutDataType=sfix(16)  OutScaling=2^0
  sync_out : Outport  Port=4  OutDataType=sfix(16)  OutScaling=2^0
  wires:
  convert_of4/2(of) -> Logical/4
  convert_of3/2(of) -> Logical/3
  convert_of2/2(of) -> Logical/2
  convert_of1/2(of) -> Logical/1
  convert_of4/1(dout) -> ri_to_c1/2
  Mux3/1 -> convert_of4/1(din)
  AddSub3/1 -> Scale3/1, Mux3/2
  Scale3/1 -> Mux3/3
  convert_of3/1(dout) -> ri_to_c1/1
  Mux2/1 -> convert_of3/1(din)
  AddSub2/1 -> Scale2/1, Mux2/2
  Scale2/1 -> Mux2/3
  convert_of2/1(dout) -> ri_to_c/2
  Mux1/1 -> convert_of2/1(din)
  AddSub1/1 -> Scale1/1, Mux1/2
  Scale1/1 -> Mux1/3
  convert_of1/1(dout) -> ri_to_c/1
  Mux/1 -> convert_of1/1(din)
  twiddle/4(bw_im) -> AddSub3/2, AddSub1/2
  twiddle/3(bw_re) -> AddSub2/2, AddSub/2
  twiddle/2(a_im) -> AddSub3/1, AddSub1/1
  twiddle/1(a_re) -> AddSub2/1, AddSub/1
  sync/1 -> twiddle/3(sync)
  b/1 -> twiddle/2(b)
  a/1 -> twiddle/1(a)
  ri_to_c/1 -> a+bw/1
  ri_to_c1/1 -> a-bw/1
  Delay/1 -> sync_out/1
  AddSub/1 -> Mux/2, Scale/1
  shift/1 -> Delay3/1
  Scale/1 -> Mux/3
  Delay3/1 -> Mux3/1, Mux2/1, Mux1/1, Mux/1
  Logical/1 -> of/1
  twiddle/5(sync_out) -> Delay/1
